simulink model "TimingTest"  (R2026b)
settings: Solver=ode4  StopTime=fixtureCfg.Duration  FixedStep=experimentCfg.Step
PostLoadFcn:
  | addpath(fullfile(fileparts(fileparts(fileparts(fileparts(fileparts(get_param(bdroot,'FileName')))))),'docs','scripts'));initialize_motor_paths();initialize_motor_model(bdroot);
model workspace (MAT data in the model file):
  currentCfg.Ts = 0.0001
  currentCfg.BandwidthHz = 500
  currentCfg.Kpd = 3.14159265359
  currentCfg.Kpq = 3.76991118431
  currentCfg.Kid = 1570.79632679
  currentCfg.Kiq = 1570.79632679
  currentCfg.Kaw = 1000
  deadtimeCfg.DeadTime = 2e-06
  deadtimeCfg.DeviceDrop = 0
  deadtimeCfg.CurrentBlend = 0.1
  deadtimeCfg.ModelEnable = 0
  deadtimeCfg.CompensationEnable = 0
  deadtimeCfg.CompensationScale = 1
  deadtimeCfg.SwitchingStep = 1e-07
  experimentCfg.Step = 5e-06
  experimentCfg.LogTs = 0.0001
  experimentCfg.Duration = 1.5
  experimentCfg.Mode = 2
  experimentCfg.UseInverter = 1
  experimentCfg.UseTiming = 1
  experimentCfg.UseMechanical = 1
  experimentCfg.ImposedElectricalSpeed = 0
  experimentCfg.IdReference = 0
  experimentCfg.IqReference = 2
  experimentCfg.IqInitial = 0
  experimentCfg.SpeedReference = 40
  experimentCfg.SpeedInitial = 0
  experimentCfg.PositionReference = 1
  experimentCfg.PositionInitial = 0
  experimentCfg.CommandTime = 0.05
  experimentCfg.LoadTorque = 0.1
  experimentCfg.LoadTime = 0.35
  experimentCfg.Enable = 1
  experimentCfg.Reset = 0
  feedforwardCfg.Enable = 0
  feedforwardCfg.ParameterScale = 1
  fixtureCfg.Ts = 0.0001
  fixtureCfg.Duration = 0.03
  fixtureCfg.SolverStep = 5e-06
  fixtureCfg.FirstStepTime = 0.003
  fixtureCfg.FirstAmplitude = 1
  fixtureCfg.SecondStepTime = 0.005
  fixtureCfg.SecondAmplitude = 2
  fixtureCfg.Inputs = [0  0; 0  0; 0  0; 0  0; 0  0; 0  0; 0  0; 0  0; 0  0; 0  0; 0  0; 0  0; 0  0; 0  0; 0  0; 0  0; 0  0; 0  0; 0  0; 0  0; 0  0; 0  0; 0  0; 0  0; 0  0; 0  0; 0  0; 0  0; 0  0; 0  0; 1  0; 1  0; 1  0; 1  0; 1  0; 1  0; 1  0; 1  0; 1  0; 1  0; 1  0; 1  0; 1  0; 1  0; 1  0; 1  0; 1  0; 1  0; 1  0; 1  0; 1  2; 1  2; 1  2; 1  2; 1  2; 1  2; 1  2; 1  2; 1  2; 1  2; 1  2; 1  2; 1  2; 1  2; 1  2; 1  2; 1  2; 1  2; 1  2; 1  2; 1  2; 1  2; 1  2; 1  2; 1  2; 1  2; 1  2; 1  2; 1  2; 1  2; 1  2; 1  2; 1  2; 1  2; 1  2; 1  2; 1  2; 1  2; 1  2; 1  2; 1  2; 1  2; 1  2; 1  2; 1  2; 1  2; 1  2; 1  2; 1  2; 1  2; 1  2; 1  2; 1  2; 1  2; 1  2; 1  2; 1  2; 1  2; 1  2; 1  2; 1  2; 1  2; 1  2; 1  2; 1  2; 1  2; 1  2; 1  2; 1  2; 1  2; 1  2; 1  2; 1  2; 1  2; 1  2; 1  2; 1  2; 1  2; 1  2; 1  2; 1  2; 1  2; 1  2; 1  2; 1  2; 1  2; 1  2; 1  2; 1  2; 1  2; 1  2; 1  2; 1  2; 1  2; 1  2; 1  2; 1  2; 1  2; 1  2; 1  2; 1  2; 1  2; 1  2; 1  2; 1  2; 1  2; 1  2; 1  2; 1  2; 1  2; 1  2; 1  2; 1  2; 1  2; 1  2; 1  2; 1  2; 1  2; 1  2; 1  2; 1  2; 1  2; 1  2; 1  2; 1  2; 1  2; 1  2; 1  2; 1  2; 1  2; 1  2; 1  2; 1  2; 1  2; 1  2; 1  2; 1  2; 1  2; 1  2; 1  2; 1  2; 1  2; 1  2; 1  2; 1  2; 1  2; 1  2; 1  2; 1  2; 1  2; 1  2; 1  2; 1  2; 1  2; 1  2; 1  2; 1  2; 1  2; 1  2; 1  2; 1  2; 1  2; 1  2; 1  2; 1  2; 1  2; 1  2; 1  2; 1  2; 1  2; 1  2; 1  2; 1  2; 1  2; 1  2; 1  2; 1  2; 1  2; 1  2; 1  2; 1  2; 1  2; 1  2; 1  2; 1  2; 1  2; 1  2; 1  2; 1  2; 1  2; 1  2; 1  2; 1  2; 1  2; 1  2; 1  2; 1  2; 1  2; 1  2; 1  2; 1  2; 1  2; 1  2; 1  2; 1  2; 1  2; 1  2; 1  2; 1  2; 1  2; 1  2; 1  2; 1  2; 1  2; 1  2; 1  2; 1  2; 1  2; 1  2; 1  2; 1  2; 1  2; 1  2; 1  2; 1  2; 1  2; 1  2; 1  2; 1  2; 1  2; 1  2; 1  2; 1  2; 1  2; 1  2; 1  2; 1  2; 1  2; 1  2; 1  2; 1  2; 1  2; 1  2; 1  2; 1  2; 1  2; 1  2; 1  2; 1  2; 1  2; 1  2]
  inverterCfg.Vdc = 48
  inverterCfg.MinDuty = 0.02
  inverterCfg.PwmTs = 0.0001
  inverterCfg.LinearLimit = 26.6043004043
  motionCfg.Ts = 0.001
  motionCfg.NaturalFrequency = 20
  motionCfg.Damping = 0.9
  motionCfg.Kt = 0.21
  motionCfg.Kp = 0.0852380952381
  motionCfg.Ki = 0.952380952381
  motionCfg.Kaw = 20
  motionCfg.PositionKp = 8
  motionCfg.SpeedLimit = 80
  motionCfg.AccelerationLimit = 200
  motionCfg.CurrentLimit = 8
  pmsmCfg.Rs = 0.5
  pmsmCfg.Ld = 0.001
  pmsmCfg.Lq = 0.0012
  pmsmCfg.Flux = 0.035
  pmsmCfg.PolePairs = 4
  pmsmCfg.J = 0.0005
  pmsmCfg.B = 0.0001
  pmsmCfg.Id0 = 0
  pmsmCfg.Iq0 = 0
  pmsmCfg.Speed0 = 0
  pmsmCfg.Position0 = 0
  testStim.time = []
  testStim.signals.values = [0  0; 0  0; 0  0; 0  0; 0  0; 0  0; 0  0; 0  0; 0  0; 0  0; 0  0; 0  0; 0  0; 0  0; 0  0; 0  0; 0  0; 0  0; 0  0; 0  0; 0  0; 0  0; 0  0; 0  0; 0  0; 0  0; 0  0; 0  0; 0  0; 0  0; 1  0; 1  0; 1  0; 1  0; 1  0; 1  0; 1  0; 1  0; 1  0; 1  0; 1  0; 1  0; 1  0; 1  0; 1  0; 1  0; 1  0; 1  0; 1  0; 1  0; 1  2; 1  2; 1  2; 1  2; 1  2; 1  2; 1  2; 1  2; 1  2; 1  2; 1  2; 1  2; 1  2; 1  2; 1  2; 1  2; 1  2; 1  2; 1  2; 1  2; 1  2; 1  2; 1  2; 1  2; 1  2; 1  2; 1  2; 1  2; 1  2; 1  2; 1  2; 1  2; 1  2; 1  2; 1  2; 1  2; 1  2; 1  2; 1  2; 1  2; 1  2; 1  2; 1  2; 1  2; 1  2; 1  2; 1  2; 1  2; 1  2; 1  2; 1  2; 1  2; 1  2; 1  2; 1  2; 1  2; 1  2; 1  2; 1  2; 1  2; 1  2; 1  2; 1  2; 1  2; 1  2; 1  2; 1  2; 1  2; 1  2; 1  2; 1  2; 1  2; 1  2; 1  2; 1  2; 1  2; 1  2; 1  2; 1  2; 1  2; 1  2; 1  2; 1  2; 1  2; 1  2; 1  2; 1  2; 1  2; 1  2; 1  2; 1  2; 1  2; 1  2; 1  2; 1  2; 1  2; 1  2; 1  2; 1  2; 1  2; 1  2; 1  2; 1  2; 1  2; 1  2; 1  2; 1  2; 1  2; 1  2; 1  2; 1  2; 1  2; 1  2; 1  2; 1  2; 1  2; 1  2; 1  2; 1  2; 1  2; 1  2; 1  2; 1  2; 1  2; 1  2; 1  2; 1  2; 1  2; 1  2; 1  2; 1  2; 1  2; 1  2; 1  2; 1  2; 1  2; 1  2; 1  2; 1  2; 1  2; 1  2; 1  2; 1  2; 1  2; 1  2; 1  2; 1  2; 1  2; 1  2; 1  2; 1  2; 1  2; 1  2; 1  2; 1  2; 1  2; 1  2; 1  2; 1  2; 1  2; 1  2; 1  2; 1  2; 1  2; 1  2; 1  2; 1  2; 1  2; 1  2; 1  2; 1  2; 1  2; 1  2; 1  2; 1  2; 1  2; 1  2; 1  2; 1  2; 1  2; 1  2; 1  2; 1  2; 1  2; 1  2; 1  2; 1  2; 1  2; 1  2; 1  2; 1  2; 1  2; 1  2; 1  2; 1  2; 1  2; 1  2; 1  2; 1  2; 1  2; 1  2; 1  2; 1  2; 1  2; 1  2; 1  2; 1  2; 1  2; 1  2; 1  2; 1  2; 1  2; 1  2; 1  2; 1  2; 1  2; 1  2; 1  2; 1  2; 1  2; 1  2; 1  2; 1  2; 1  2; 1  2; 1  2; 1  2; 1  2; 1  2; 1  2; 1  2; 1  2; 1  2; 1  2; 1  2; 1  2; 1  2; 1  2; 1  2; 1  2; 1  2; 1  2; 1  2; 1  2; 1  2; 1  2; 1  2; 1  2; 1  2; 1  2; 1  2]
  testStim.signals.dimensions = 2
  timingCfg.Ts = 0.0001
  timingCfg.FeedbackTicks = 1
  timingCfg.ActuationTicks = 1
libraries: ControlTiming x2
settings Model: Creator=24322  LastModifiedBy=24322

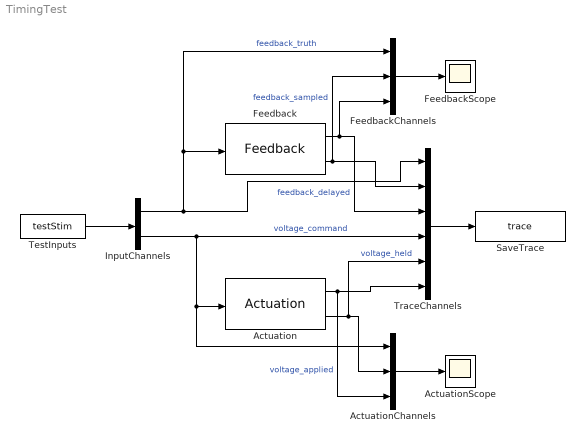
== system TimingTest ==
  Actuation : ControlTiming/Actuation  SystemSampleTime=-1  VariantActivationTime=update diagram  EmptyChoice=off  PassThrough=off  PassThroughVariantControl=(default)  EmptyChoiceVariantControl=(default)  AllowFlexibleInterface=on  Latency=0  AutoFrameSizeCalculation=off
  ActuationChannels : Mux  Inputs=3
  ActuationScope : Scope
      settings: Title=Actuation  YLabel=V
  Feedback : ControlTiming/Feedback  SystemSampleTime=-1  VariantActivationTime=update diagram  EmptyChoice=off  PassThrough=off  PassThroughVariantControl=(default)  EmptyChoiceVariantControl=(default)  AllowFlexibleInterface=on  Latency=0  AutoFrameSizeCalculation=off
  FeedbackChannels : Mux  Inputs=3
  FeedbackScope : Scope
      settings: Title=Feedback  YLabel=1
  InputChannels : Demux  Outputs=2
  SaveTrace : ToWorkspace  VariableName=trace  SaveFormat=Structure With Time  SampleTime=experimentCfg.LogTs
  TestInputs : FromWorkspace  VariableName=testStim  SampleTime=currentCfg.Ts  Interpolate=off  OutputAfterFinalValue=Holding final value
  TraceChannels : Mux  Inputs=6
  wires:
  TraceChannels/1 -> SaveTrace/1
  TestInputs/1 -> InputChannels/1
  ActuationChannels/1 -> ActuationScope/1
  FeedbackChannels/1 -> FeedbackScope/1
  InputChannels/1 -> FeedbackChannels/1, Feedback/1, TraceChannels/1  "feedback_truth"
  InputChannels/2 -> ActuationChannels/1, Actuation/1, TraceChannels/4  "voltage_command"
  Feedback/2 -> FeedbackChannels/2, TraceChannels/2  "feedback_sampled"
  Feedback/1 -> FeedbackChannels/3, TraceChannels/3  "feedback_delayed"
  Actuation/2 -> ActuationChannels/2, TraceChannels/5  "voltage_held"
  Actuation/1 -> ActuationChannels/3, TraceChannels/6  "voltage_applied"
